simulink model "FMS"  (R2018b)
settings: configuration reference "fms_config" (kept outside this file)
values from neighbouring files (symbols this model uses):
  FMS_EXPORT = Simulink.Parameter(FMS_EXPORT_VALUE)    [fms_model_init.m]
  FMS_PARAM = Simulink.Parameter(FMS_PARAM_VALUE)    [fms_model_init.m]
undefined symbols (not defined in the file or in its folder): actuator_cmd, cmd_mask, ControlMode, ctrl_mode, DiscIntNeverNeededParam, FMS_Cmd, home, mode, PilotMode, r_cmd, reset, state, status, timestamp, u_cmd, VehicleState, VehicleStatus, wp_consume, wp_current
libraries: simulink x46, FMT_Model_Lib x35, hdlsllib x2
(part 2 of 3)

== system FMS/FMS Commander/Commander/Arm/Assist/Position/Velocity_Command/DeadZone ==
  u : Inport
  Dead Zone : DeadZone  LowerValue=-th  UpperValue=th  SaturateOnIntegerOverflow=on
  Gain : Gain  Gain=1/(1-th)
  y : Outport
  wires:
  Gain/1 -> y/1
  Dead Zone/1 -> Gain/1
  u/1 -> Dead Zone/1

== system FMS/FMS Commander/Commander/Arm/Assist/Stabilize/Heading Command/Controller ==
  motion_state : Inport
  In Bus Element : Inport  Port=2  PortName=FMS_In
  In Bus Element1 : Inport  Port=2  PortName=FMS_In
  Brake Control : Subsystem  TreatAsAtomicUnit=on
  Hold Control : Subsystem  TreatAsAtomicUnit=on
  Merge : Merge  Inputs=3
  Move Control : Subsystem  TreatAsAtomicUnit=on
  Switch Case : SwitchCase  CaseConditions={MotionState.Hold, MotionState.Brake, MotionState.Move}  ShowDefaultCase=off
  psi_rate_cmd_radPs : Outport
  wires:
  Move Control/1(psi_rate_cmd_radPs) -> Merge/3
  Hold Control/1(psi_rate_cmd_radPs) -> Merge/1
  In Bus Element/1 -> Hold Control/1(FMS_In)
  Switch Case/1 -> Hold Control/Action
  motion_state/1 -> Switch Case/1
  In Bus Element1/1 -> Move Control/1(FMS_In)
  Merge/1 -> psi_rate_cmd_radPs/1
  Switch Case/3 -> Move Control/Action
  Brake Control/1(psi_rate_cmd_radPs) -> Merge/2
  Switch Case/2 -> Brake Control/Action

== system FMS/FMS Commander/Commander/Arm/Assist/Stabilize/Heading Command/Detect Movement ==
  FMS_In : Inport
  Abs1 : Abs
  Abs2 : Abs
  Bus Selector1 : BusSelector  OutputSignals=Pilot_Cmd.stick_roll,Pilot_Cmd.stick_throttle
  Compare To Constant : simulink/Logic and Bit Operations/Compare To Constant  relop=>  const=0.1  OutDataTypeStr=boolean
  Compare To Constant1 : simulink/Logic and Bit Operations/Compare To Constant  relop=<=  const=0.15  OutDataTypeStr=boolean
  Logical Operator : Logic  Operator=OR  AllPortsSameDT=off  OutDataTypeStr=boolean
  Motion State : Stateflow chart  TreatAsAtomicUnit=on
  motion_state : Outport
  wires:
  FMS_In/1 -> Bus Selector1/1
  Compare To Constant/1 -> Logical Operator/1
  Abs1/1 -> Compare To Constant/1
  Motion State/1(state) -> motion_state/1  "pos_ms"
  Bus Selector1/1 -> Abs1/1  "<stick_roll>"
  Bus Selector1/2 -> Abs2/1  "<stick_throttle>"
  Abs2/1 -> Compare To Constant1/1
  Compare To Constant1/1 -> Logical Operator/2
  Logical Operator/1 -> Motion State/1(motion_req)

== system FMS/FMS Commander/Commander/Arm/Assist/Stabilize/Reset/DeadZone ==
  u : Inport
  Dead Zone : DeadZone  LowerValue=-th  UpperValue=th  SaturateOnIntegerOverflow=on
  Gain : Gain  Gain=1/(1-th)
  y : Outport
  wires:
  Gain/1 -> y/1
  Dead Zone/1 -> Gain/1
  u/1 -> Dead Zone/1

== system FMS/FMS Commander/Commander/Arm/Assist/Stabilize/Reset/DeadZone1 ==
  u : Inport
  Dead Zone : DeadZone  LowerValue=-th  UpperValue=th  SaturateOnIntegerOverflow=on
  Gain : Gain  Gain=1/(1-th)
  y : Outport
  wires:
  u/1 -> Dead Zone/1
  Dead Zone/1 -> Gain/1
  Gain/1 -> y/1

== system FMS/FMS Commander/Commander/Arm/Auto/Mission/Mission_SubSystem/Velocity Commander ==
  p1 : Inport
  p2 : Inport  Port=2
  p3 : Inport  Port=3
  L1 : Inport  Port=4
  In Bus Element : Inport  Port=5  PortName=FMS_In  Element=INS_Out.vn
  In Bus Element1 : Inport  Port=5  PortName=FMS_In  Element=INS_Out.ve
  AccToRate : Gain  Gain=FMS_PARAM.AY_P
  L1 Reference WP : Subsystem
  Lateral Acceleration : Subsystem
  Mux1 : Mux  Inputs=2
  r_cmd : Outport
  wires:
  p3/1 -> Lateral Acceleration/3(p3), L1 Reference WP/3(P3)
  In Bus Element1/1 -> Mux1/2
  Mux1/1 -> Lateral Acceleration/1(Vg)
  p2/1 -> L1 Reference WP/2(P2)
  Lateral Acceleration/1(l1_a_cmd) -> AccToRate/1
  In Bus Element/1 -> Mux1/1
  L1 Reference WP/1(L1_WP) -> Lateral Acceleration/2(L1_WP)  "L1_WP"
  p1/1 -> L1 Reference WP/1(P1)
  L1/1 -> L1 Reference WP/4(L1), Lateral Acceleration/4(L1)
  AccToRate/1 -> r_cmd/1

== system FMS/FMS Commander/Commander/Arm/Auto/Mission/Mission_SubSystem/Way Points ==
  note: P1: path start point
      | P2: path end point
      | P3: vehicle point
  FMS_In : Inport
  Bus Selector : BusSelector  OutputSignals=INS_Out.x_R,INS_Out.y_R
  Bus Selector1 : BusSelector  OutputSignals=Cmd_In.sp_waypoint
  Bus Selector2 : BusSelector  OutputSignals=Cmd_In.cur_waypoint
  Mux : Mux  Inputs=2
  Reshape : Reshape  OutputDimensionality=Customize  OutputDimensions=[2,1]
  Reshape1 : Reshape  OutputDimensionality=Customize  OutputDimensions=[2,1]
  Reshape2 : Reshape  OutputDimensionality=Customize  OutputDimensions=[2,1]
  Selector : Selector  InputPortWidth=3  IndexOptions=Index vector (dialog)  Indices=[1 2]  OutputSizes=1
  Selector1 : Selector  InputPortWidth=3  IndexOptions=Index vector (dialog)  Indices=[1 2]  OutputSizes=1
  p1 : Outport
  p2 : Outport  Port=2
  p3 : Outport  Port=3
  wires:
  Reshape2/1 -> p3/1
  Reshape1/1 -> p1/1
  Reshape/1 -> p2/1
  Bus Selector/2 -> Mux/2  "<y_R>"
  Bus Selector/1 -> Mux/1  "<x_R>"
  FMS_In/1 -> Bus Selector2/1, Bus Selector1/1, Bus Selector/1
  Bus Selector1/1 -> Selector/1  "<sp_waypoint>"
  Selector/1 -> Reshape/1
  Bus Selector2/1 -> Selector1/1  "<cur_waypoint>"
  Mux/1 -> Reshape2/1
  Selector1/1 -> Reshape1/1

== system FMS/FMS Commander/Commander/Arm/Auto/Offboard/Velocity Rotation Command/Heading_Control ==
  FMS_In : Inport
  Bus Selector1 : BusSelector  OutputSignals=Auto_Cmd.psi_cmd
  Bus Selector2 : BusSelector  OutputSignals=INS_Out.psi
  Gain2 : Gain  Gain=FMS_PARAM.YAW_P  OutDataTypeStr=single
  Sum : Sum  Inputs=-+|
  psi_err_saturation : Subsystem
  heading_r_cmd : Outport
  wires:
  Sum/1 -> psi_err_saturation/1(psi_err_in)  "psi_error_rad"
  psi_err_saturation/1(psi_err_rad) -> Gain2/1
  Gain2/1 -> heading_r_cmd/1
  FMS_In/1 -> Bus Selector1/1, Bus Selector2/1
  Bus Selector2/1 -> Sum/1  "<psi>"
  Bus Selector1/1 -> Sum/2  "<psi_cmd>"

== system FMS/FMS Commander/Commander/Arm/Auto/Offboard/Velocity Rotation Command/Position Data ==
  FMS_In : Inport
  Bus Selector : BusSelector  OutputSignals=INS_Out.x_R,INS_Out.y_R
  Mux : Mux  Inputs=2
  Position Command : Subsystem
  Reshape : Reshape  OutputDimensionality=Customize  OutputDimensions=[2,1]
  Reshape1 : Reshape  OutputDimensionality=Customize  OutputDimensions=[2,1]
  pos_R : Outport
  pos_cmd : Outport  Port=2
  wires:
  Reshape1/1 -> pos_R/1
  Reshape/1 -> pos_cmd/1
  Bus Selector/2 -> Mux/2  "<y_R>"
  Bus Selector/1 -> Mux/1  "<x_R>"
  FMS_In/1 -> Position Command/1(FMS_In), Bus Selector/1
  Position Command/1(pos_O_cmd) -> Reshape/1
  Mux/1 -> Reshape1/1

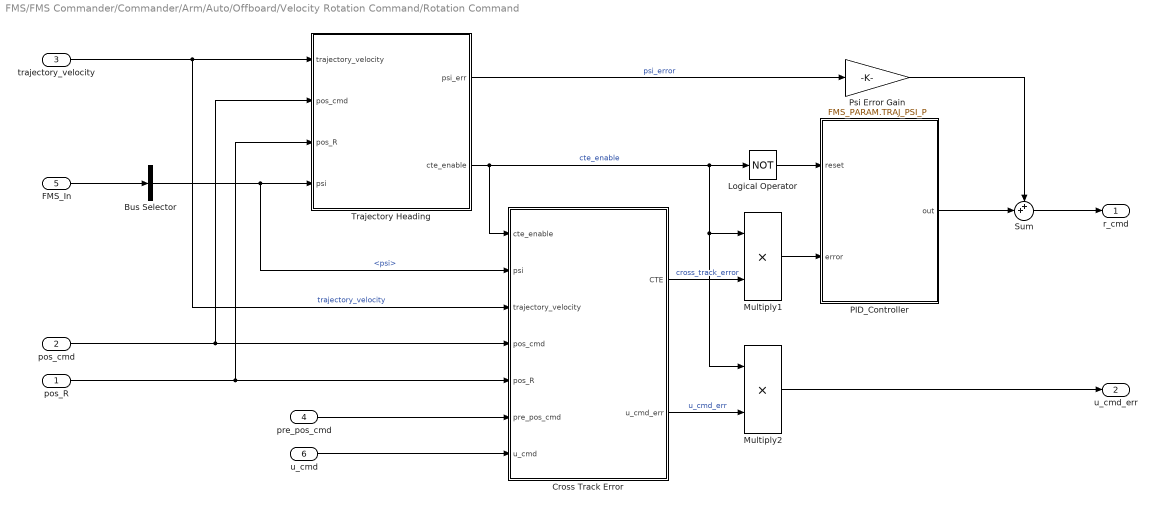
== system FMS/FMS Commander/Commander/Arm/Auto/Offboard/Velocity Rotation Command/Rotation Command ==
  pos_R : Inport
  pos_cmd : Inport  Port=2
  trajectory_velocity : Inport  Port=3
  pre_pos_cmd : Inport  Port=4
  FMS_In : Inport  Port=5
  u_cmd : Inport  Port=6
  Bus Selector : BusSelector  OutputSignals=INS_Out.psi
  Cross Track Error : Subsystem
  Logical Operator : Logic  Operator=NOT  AllPortsSameDT=off  OutDataTypeStr=boolean
  Multiply1 : Product
  Multiply2 : Product
  PID_Controller : Subsystem
  Psi Error Gain : Gain  Gain=FMS_PARAM.TRAJ_PSI_P  OutDataTypeStr=Inherit: Same as input
  Sum : Sum  Inputs=++|
  Trajectory Heading : Subsystem
  r_cmd : Outport
  u_cmd_err : Outport  Port=2
  wires:
  pos_cmd/1 -> Trajectory Heading/2(pos_cmd), Cross Track Error/4(pos_cmd)
  trajectory_velocity/1 -> Cross Track Error/3(trajectory_velocity), Trajectory Heading/1(trajectory_velocity)  "trajectory_velocity"
  pos_R/1 -> Trajectory Heading/3(pos_R), Cross Track Error/5(pos_R)
  Bus Selector/1 -> Trajectory Heading/4(psi), Cross Track Error/2(psi)  "<psi>"
  Cross Track Error/1(CTE) -> Multiply1/2  "cross_track_error"
  Psi Error Gain/1 -> Sum/1
  u_cmd/1 -> Cross Track Error/7(u_cmd)
  FMS_In/1 -> Bus Selector/1
  pre_pos_cmd/1 -> Cross Track Error/6(pre_pos_cmd)
  Cross Track Error/2(u_cmd_err) -> Multiply2/2  "u_cmd_err"
  Multiply2/1 -> u_cmd_err/1
  PID_Controller/1(out) -> Sum/2
  Sum/1 -> r_cmd/1
  Trajectory Heading/1(psi_err) -> Psi Error Gain/1  "psi_error"
  Trajectory Heading/2(cte_enable) -> Cross Track Error/1(cte_enable), Logical Operator/1, Multiply2/1, Multiply1/1  "cte_enable"
  Multiply1/1 -> PID_Controller/2(error)
  Logical Operator/1 -> PID_Controller/1(reset)

== system FMS/FMS Commander/Commander/Arm/Auto/Offboard/Velocity Rotation Command/Signal_Route ==
  FMS_In : Inport
  heading_r_cmd : Inport  Port=2
  pos_r_cmd : Inport  Port=3
  Bus Selector : BusSelector  OutputSignals=Auto_Cmd.cmd_mask
  Bus Selector1 : BusSelector  OutputSignals=Auto_Cmd.r_cmd
  Switch : Switch  Criteria=u2 > Threshold
  Switch1 : Switch  Criteria=u2 > Threshold
  psi_cmd_valid : simulink/Logic and Bit Operations/Bitwise Operator  logicop=AND  UseBitMask=on  BitMask=bin2dec('100000')  BitMaskRealWorld=Stored Integer
  r_cmd_valid : simulink/Logic and Bit Operations/Bitwise Operator  logicop=AND  UseBitMask=on  BitMask=bin2dec('100')  BitMaskRealWorld=Stored Integer
  r_cmd : Outport
  wires:
  FMS_In/1 -> Bus Selector1/1, Bus Selector/1
  pos_r_cmd/1 -> Switch1/3
  r_cmd_valid/1 -> Switch/2
  Bus Selector1/1 -> Switch/1  "<r_cmd>"
  Switch/1 -> r_cmd/1
  Bus Selector/1 -> psi_cmd_valid/1, r_cmd_valid/1  "<cmd_mask>"
  psi_cmd_valid/1 -> Switch1/2
  heading_r_cmd/1 -> Switch1/1
  Switch1/1 -> Switch/3

== system FMS/FMS Commander/Commander/Arm/Auto/Offboard/Velocity Rotation Command/Trajectory Velocity ==
  pos_cmd : Inport  OutDataTypeStr=single  PortDimensions=[2 1]
  pos_R : Inport  Port=2
  FMS_In : Inport  Port=3
  Bus Selector : BusSelector  OutputSignals=Auto_Cmd.timestamp
  Divide : Product  Inputs=*/
  Low Pass Filter : Subsystem
  Previous Pos Cmd : Subsystem
  Sum : Sum  Inputs=+-|
  dT Estimator : Subsystem
  trajectory_velocity : Outport  OutDataTypeStr=single  PortDimensions=[2 1]  VectorParamsAs1DForOutWhenUnconnected=on
  pre_pos_cmd : Outport  Port=2  OutDataTypeStr=single  PortDimensions=[2 1]  VectorParamsAs1DForOutWhenUnconnected=on
  wires:
  Low Pass Filter/1(y) -> trajectory_velocity/1
  Divide/1 -> Low Pass Filter/1(u)
  Sum/1 -> Divide/1
  pos_cmd/1 -> Sum/1, Previous Pos Cmd/1(pos_cmd)  "pos_cmd"
  pos_R/1 -> Previous Pos Cmd/2(pos_R)
  Previous Pos Cmd/1(prev_pos_cmd) -> pre_pos_cmd/1, Sum/2  "pre_pos_cmd"
  FMS_In/1 -> Bus Selector/1
  Bus Selector/1 -> dT Estimator/1(timestamp)  "<timestamp>"
  dT Estimator/1(dT) -> Divide/2  "dT"

== system FMS/FMS Commander/Commander/Arm/Auto/Offboard/Velocity Rotation Command/Velocity Command ==
  note: u command is always in body frame for car
  trajectory_velocity : Inport
  FMS_In : Inport  Port=2
  Bus Selector1 : BusSelector  OutputSignals=Auto_Cmd.cmd_mask
  Bus Selector2 : BusSelector  OutputSignals=Auto_Cmd.u_cmd
  Compare To Zero2 : simulink/Logic and Bit Operations/Compare To Zero  relop=>  OutDataTypeStr=boolean
  Saturation1 : Saturate  UpperLimit=FMS_PARAM.MAX_VEL  LowerLimit=0
  Switch : Switch  Criteria=u2 > Threshold
  Vector Modulus : FMT_Model_Lib/Math/Vector Modulus
      settings: SourceProductName=FMT Toolbox
  u_cmd valid : simulink/Logic and Bit Operations/Bitwise Operator  logicop=AND  UseBitMask=on  BitMask=bin2dec('10000000000000')  BitMaskRealWorld=Stored Integer
  u_cmd_C : Outport
  wires:
  Compare To Zero2/1 -> Switch/2
  Bus Selector2/1 -> Switch/1  "<u_cmd>"
  Saturation1/1 -> Switch/3
  Switch/1 -> u_cmd_C/1
  Bus Selector1/1 -> u_cmd valid/1  "<cmd_mask>"
  u_cmd valid/1 -> Compare To Zero2/1
  FMS_In/1 -> Bus Selector1/1, Bus Selector2/1
  trajectory_velocity/1 -> Vector Modulus/1
  Vector Modulus/1 -> Saturation1/1  "trajectory_speed"

== system FMS/FMS Commander/Commander/Arm/SubMode/Return/Velocity Commander/L1 Reference WP ==
  P1 : Inport
  P2 : Inport  Port=2
  P3 : Inport  Port=3
  L1 : Inport  Port=4
  Compare To Constant : simulink/Logic and Bit Operations/Compare To Constant  relop=>=  const=0  OutDataTypeStr=boolean
  Compare To Constant1 : simulink/Logic and Bit Operations/Compare To Constant  relop=>  const=0  OutDataTypeStr=boolean
  NearbyRefWP : MATLAB Function  TreatAsAtomicUnit=on
  OutRegionRegWP : MATLAB Function  TreatAsAtomicUnit=on
  Reshape : Reshape  OutputDimensionality=Customize  OutputDimensions=[2,1]
  SearchL1RefWP : MATLAB Function  TreatAsAtomicUnit=on
  Switch : Switch  Criteria=u2 > Threshold
  Switch1 : Switch  Criteria=u2 > Threshold
  L1_WP : Outport
  wires:
  Reshape/1 -> L1_WP/1
  Compare To Constant/1 -> Switch/2
  NearbyRefWP/2(d) -> Compare To Constant1/1  "distance"
  SearchL1RefWP/2(u) -> Compare To Constant/1  "l1_u"
  Compare To Constant1/1 -> Switch1/2
  P1/1 -> SearchL1RefWP/1(P1), OutRegionRegWP/1(P1)
  P2/1 -> SearchL1RefWP/2(P2), NearbyRefWP/1(P2), OutRegionRegWP/2(P2)
  P3/1 -> NearbyRefWP/2(P3), SearchL1RefWP/3(P3), OutRegionRegWP/3(P3)
  Switch/1 -> Switch1/3
  L1/1 -> SearchL1RefWP/4(L1), NearbyRefWP/3(L1)
  OutRegionRegWP/1(P) -> Switch/3  "out_WP"
  Switch1/1 -> Reshape/1
  SearchL1RefWP/1(P) -> Switch/1  "L1_Ref_P"
  NearbyRefWP/1(P) -> Switch1/1  "NearbyWP"

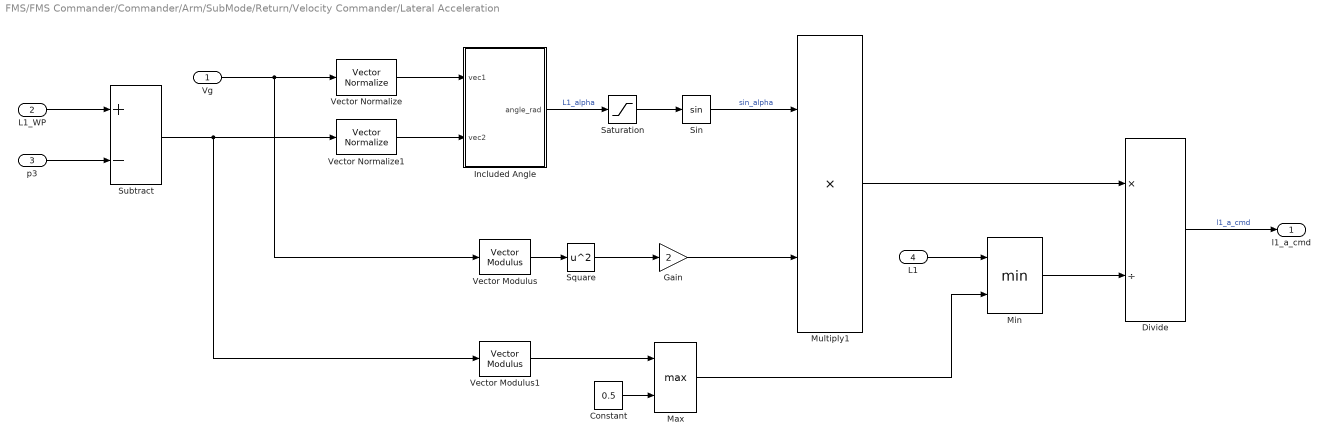
== system FMS/FMS Commander/Commander/Arm/SubMode/Return/Velocity Commander/Lateral Acceleration ==
  Vg : Inport
  L1_WP : Inport  Port=2
  p3 : Inport  Port=3
  L1 : Inport  Port=4
  Constant : Constant  Value=0.5  OutDataTypeStr=Inherit: Inherit via back propagation
  Divide : Product  Inputs=*/
  Gain : Gain  Gain=2
  Included Angle : Subsystem
  Max : MinMax  Function=max  Inputs=2
  Min : MinMax  Inputs=2
  Multiply1 : Product
  Saturation : Saturate  UpperLimit=pi/2  LowerLimit=-pi/2
  Sin : Trigonometry
  Square : Math  Operator=square  SaturateOnIntegerOverflow=on
  Subtract : Sum  Inputs=+-
  Vector Modulus : FMT_Model_Lib/Math/Vector Modulus
      settings: SourceProductName=FMT Toolbox
  Vector Modulus1 : FMT_Model_Lib/Math/Vector Modulus
      settings: SourceProductName=FMT Toolbox
  Vector Normalize : FMT_Model_Lib/Math/Vector Normalize
      settings: SourceProductName=FMT Toolbox
  Vector Normalize1 : FMT_Model_Lib/Math/Vector Normalize
      settings: SourceProductName=FMT Toolbox
  l1_a_cmd : Outport
  wires:
  Saturation/1 -> Sin/1
  Included Angle/1(angle_rad) -> Saturation/1  "L1_alpha"
  Vector Modulus/1 -> Square/1
  Subtract/1 -> Vector Modulus1/1, Vector Normalize1/1
  Gain/1 -> Multiply1/2
  L1_WP/1 -> Subtract/1
  Vector Normalize/1 -> Included Angle/1(vec1)
  Multiply1/1 -> Divide/1
  Divide/1 -> l1_a_cmd/1  "l1_a_cmd"
  Vector Normalize1/1 -> Included Angle/2(vec2)
  Square/1 -> Gain/1
  L1/1 -> Min/1
  Vg/1 -> Vector Normalize/1, Vector Modulus/1
  Sin/1 -> Multiply1/1  "sin_alpha"
  p3/1 -> Subtract/2
  Vector Modulus1/1 -> Max/1
  Constant/1 -> Max/2
  Max/1 -> Min/2
  Min/1 -> Divide/2

== system FMS/FMS Commander/Commander/Arm/Assist/Position/Position Command/Controller/Brake Control ==
  Action Port : ActionPort  InitializeStates=reset  ActionType=case
  Constant : Constant  Value=0  OutDataTypeStr=single
  r_cmd_radPs : Outport
  wires:
  Constant/1 -> r_cmd_radPs/1

== system FMS/FMS Commander/Commander/Arm/Assist/Position/Position Command/Controller/Hold Control ==
  FMS_In : Inport
  u_cmd : Inport  Port=2
  Action Port : ActionPort  InitializeStates=reset  ActionType=case
  AccToRate : Gain  Gain=FMS_PARAM.AY_P
  Bus Selector1 : BusSelector  OutputSignals=INS_Out.vn,INS_Out.ve
  FMS_In1 : InportShadow
  L1 : Constant  Value=FMS_PARAM.L1  OutDataTypeStr=single
  L1_Reference_WP : Subsystem
  Lateral_Acceleration : Subsystem
  Mux : Mux  Inputs=2
  Path_Ray : Subsystem
  r_cmd_radPs : Outport
  wires:
  FMS_In/1 -> Path_Ray/1(FMS_In)
  Path_Ray/1(p_vehicle) -> Lateral_Acceleration/1(p_vehicle), L1_Reference_WP/1(c)
  Path_Ray/2(p_0) -> L1_Reference_WP/2(p_0)
  Path_Ray/3(n) -> L1_Reference_WP/3(n)
  L1/1 -> L1_Reference_WP/4(L1), Lateral_Acceleration/3(L1)
  FMS_In1/1 -> Bus Selector1/1
  Bus Selector1/1 -> Mux/1  "<vn>"
  Bus Selector1/2 -> Mux/2  "<ve>"
  L1_Reference_WP/1(L1_WP) -> Lateral_Acceleration/2(L1_WP)
  Mux/1 -> Lateral_Acceleration/4(Vg)
  Lateral_Acceleration/1(ay_cmd_mPs2) -> AccToRate/1
  AccToRate/1 -> r_cmd_radPs/1
  u_cmd/1 -> Path_Ray/2(u_cmd)

== system FMS/FMS Commander/Commander/Arm/Assist/Position/Position Command/Controller/Move Control ==
  FMS_In : Inport
  Action Port : ActionPort  InitializeStates=reset  ActionType=case
  Bus Selector : BusSelector  OutputSignals=Pilot_Cmd.stick_roll
  DeadZone : Subsystem  mask{th=0.1}
      mask prompts: th "Threshold"
      mask Display: disp('Dead Zone')
  Gain6 : Gain  Gain=FMS_PARAM.MAX_R  OutDataTypeStr=single
  r_cmd_radPs : Outport
  wires:
  Bus Selector/1 -> DeadZone/1(u)  "<stick_roll>"
  Gain6/1 -> r_cmd_radPs/1
  FMS_In/1 -> Bus Selector/1
  DeadZone/1(y) -> Gain6/1

== system FMS/FMS Commander/Commander/Arm/Assist/Stabilize/Heading Command/Controller/Brake Control ==
  Action Port : ActionPort  InitializeStates=reset  ActionType=case
  Constant : Constant  Value=0  OutDataTypeStr=single
  psi_rate_cmd_radPs : Outport
  wires:
  Constant/1 -> psi_rate_cmd_radPs/1

== system FMS/FMS Commander/Commander/Arm/Assist/Stabilize/Heading Command/Controller/Hold Control ==
  FMS_In : Inport
  Action Port : ActionPort  InitializeStates=reset  ActionType=case
  Bus_Selection : Subsystem
  Delay : Delay  DelayLength=1  InitialConditionSource=Input port
      settings: InputPortMap=u0,p4
  Gain2 : Gain  Gain=FMS_PARAM.YAW_P  OutDataTypeStr=single
  Sum : Sum  Inputs=-+|
  psi_err_saturation : Subsystem
  psi_rate_cmd_radPs : Outport
  wires:
  FMS_In/1 -> Bus_Selection/1(FMS_In)
  Gain2/1 -> psi_rate_cmd_radPs/1
  psi_err_saturation/1(psi_err_rad) -> Gain2/1
  Sum/1 -> psi_err_saturation/1(psi_err_in)  "psi_error_rad"
  Delay/1 -> Sum/2, Delay/1  "psi_cmd_rad"
  Bus_Selection/1(psi_rad) -> Delay/2, Sum/1  "psi_est_rad"

== system FMS/FMS Commander/Commander/Arm/Assist/Stabilize/Heading Command/Controller/Move Control ==
  FMS_In : Inport
  Action Port : ActionPort  InitializeStates=reset  ActionType=case
  Bus Selector : BusSelector  OutputSignals=Pilot_Cmd.stick_roll
  DeadZone : Subsystem  mask{th=0.1}
      mask prompts: th "Threshold"
      mask Display: disp('Dead Zone')
  Gain : Gain  Gain=FMS_PARAM.MAX_R
  psi_rate_cmd_radPs : Outport
  wires:
  Bus Selector/1 -> DeadZone/1(u)  "<stick_roll>"
  FMS_In/1 -> Bus Selector/1
  DeadZone/1(y) -> Gain/1
  Gain/1 -> psi_rate_cmd_radPs/1

== system FMS/FMS Commander/Commander/Arm/Auto/Mission/Mission_SubSystem/Velocity Commander/L1 Reference WP ==
  P1 : Inport
  P2 : Inport  Port=2
  P3 : Inport  Port=3
  L1 : Inport  Port=4
  Compare To Constant : simulink/Logic and Bit Operations/Compare To Constant  relop=>=  const=0  OutDataTypeStr=boolean
  Compare To Constant1 : simulink/Logic and Bit Operations/Compare To Constant  relop=>  const=0  OutDataTypeStr=boolean
  NearbyRefWP : MATLAB Function  TreatAsAtomicUnit=on
  OutRegionRegWP : MATLAB Function  TreatAsAtomicUnit=on
  Reshape : Reshape  OutputDimensionality=Customize  OutputDimensions=[2,1]
  SearchL1RefWP : MATLAB Function  TreatAsAtomicUnit=on
  Switch : Switch  Criteria=u2 > Threshold
  Switch1 : Switch  Criteria=u2 > Threshold
  L1_WP : Outport
  wires:
  Reshape/1 -> L1_WP/1
  Compare To Constant/1 -> Switch/2
  NearbyRefWP/2(d) -> Compare To Constant1/1  "distance"
  SearchL1RefWP/2(u) -> Compare To Constant/1  "l1_u"
  Compare To Constant1/1 -> Switch1/2
  P1/1 -> SearchL1RefWP/1(P1), OutRegionRegWP/1(P1)
  P2/1 -> SearchL1RefWP/2(P2), NearbyRefWP/1(P2), OutRegionRegWP/2(P2)
  P3/1 -> NearbyRefWP/2(P3), SearchL1RefWP/3(P3), OutRegionRegWP/3(P3)
  Switch/1 -> Switch1/3
  L1/1 -> SearchL1RefWP/4(L1), NearbyRefWP/3(L1)
  OutRegionRegWP/1(P) -> Switch/3  "out_WP"
  Switch1/1 -> Reshape/1
  SearchL1RefWP/1(P) -> Switch/1  "L1_Ref_P"
  NearbyRefWP/1(P) -> Switch1/1  "NearbyWP"

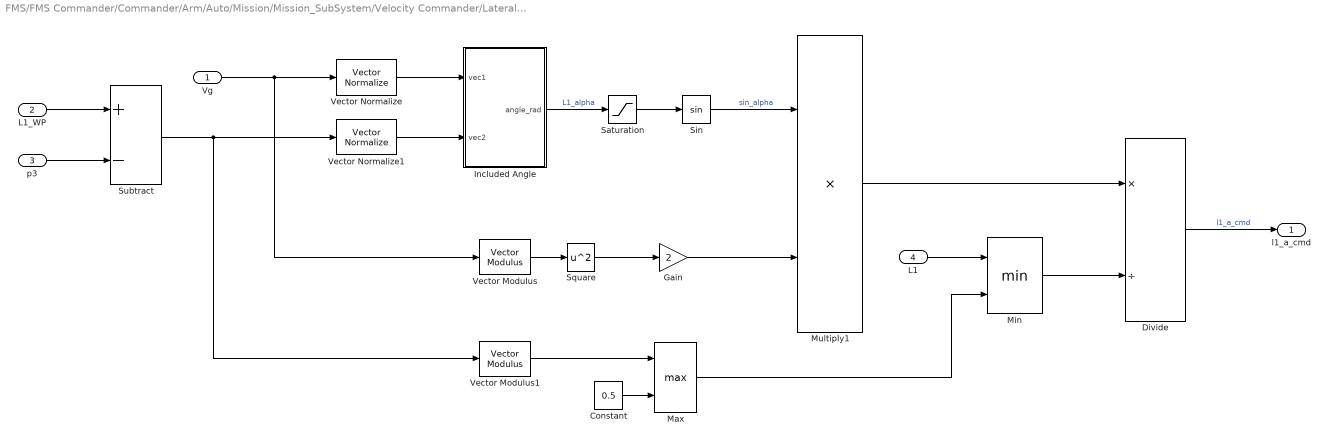
== system FMS/FMS Commander/Commander/Arm/Auto/Mission/Mission_SubSystem/Velocity Commander/Lateral Acceleration ==
  Vg : Inport
  L1_WP : Inport  Port=2
  p3 : Inport  Port=3
  L1 : Inport  Port=4
  Constant : Constant  Value=0.5  OutDataTypeStr=Inherit: Inherit via back propagation
  Divide : Product  Inputs=*/
  Gain : Gain  Gain=2
  Included Angle : Subsystem
  Max : MinMax  Function=max  Inputs=2
  Min : MinMax  Inputs=2
  Multiply1 : Product
  Saturation : Saturate  UpperLimit=pi/2  LowerLimit=-pi/2
  Sin : Trigonometry
  Square : Math  Operator=square  SaturateOnIntegerOverflow=on
  Subtract : Sum  Inputs=+-
  Vector Modulus : FMT_Model_Lib/Math/Vector Modulus
      settings: SourceProductName=FMT Toolbox
  Vector Modulus1 : FMT_Model_Lib/Math/Vector Modulus
      settings: SourceProductName=FMT Toolbox
  Vector Normalize : FMT_Model_Lib/Math/Vector Normalize
      settings: SourceProductName=FMT Toolbox
  Vector Normalize1 : FMT_Model_Lib/Math/Vector Normalize
      settings: SourceProductName=FMT Toolbox
  l1_a_cmd : Outport
  wires:
  Saturation/1 -> Sin/1
  Included Angle/1(angle_rad) -> Saturation/1  "L1_alpha"
  Vector Modulus/1 -> Square/1
  Subtract/1 -> Vector Modulus1/1, Vector Normalize1/1
  Gain/1 -> Multiply1/2
  L1_WP/1 -> Subtract/1
  Vector Normalize/1 -> Included Angle/1(vec1)
  Multiply1/1 -> Divide/1
  Divide/1 -> l1_a_cmd/1  "l1_a_cmd"
  Vector Normalize1/1 -> Included Angle/2(vec2)
  Square/1 -> Gain/1
  L1/1 -> Min/1
  Vg/1 -> Vector Normalize/1, Vector Modulus/1
  Sin/1 -> Multiply1/1  "sin_alpha"
  p3/1 -> Subtract/2
  Vector Modulus1/1 -> Max/1
  Constant/1 -> Max/2
  Max/1 -> Min/2
  Min/1 -> Divide/2

== system FMS/FMS Commander/Commander/Arm/Auto/Offboard/Velocity Rotation Command/Heading_Control/psi_err_saturation ==
  psi_err_in : Inport
  Abs : Abs
  Compare To Constant : simulink/Logic and Bit Operations/Compare To Constant  relop=>  const=pi  OutDataTypeStr=boolean
  Constant : Constant  Value=2*pi  OutDataTypeStr=single
  Multiply : Product
  Sign : Signum
  Subtract : Sum  Inputs=-+
  Switch : Switch  Criteria=u2 > Threshold
  psi_err_rad : Outport
  wires:
  Multiply/1 -> Switch/1
  Sign/1 -> Multiply/2
  Subtract/1 -> Multiply/1
  Constant/1 -> Subtract/1
  Switch/1 -> psi_err_rad/1
  Compare To Constant/1 -> Switch/2
  Abs/1 -> Compare To Constant/1, Subtract/2
  psi_err_in/1 -> Abs/1, Switch/3, Sign/1

== system FMS/FMS Commander/Commander/Arm/Auto/Offboard/Velocity Rotation Command/Position Data/Position Command ==
  FMS_In : Inport
  Body_FRD : Subsystem
  Bus Selector : BusSelector  OutputSignals=INS_Out
  Bus Selector2 : BusSelector  OutputSignals=Auto_Cmd.frame
  Command_Mask : Subsystem
  Global_NED : Subsystem
  Index Vector : MultiPortSwitch  DataPortOrder=Zero-based contiguous  Inputs=4  zeroidx=on
  Local_FRD : Subsystem
  Local_NED : Subsystem
  Position_Command : Subsystem
  Selector : Selector  InputPortWidth=3  IndexOptions=Index vector (dialog)  Indices=[1 2]  OutputSizes=1
  pos_O_cmd : Outport
  wires:
  Position_Command/1(pos_cmd_R) -> Local_FRD/1(pos_R_cmd), Body_FRD/2(pos_B_cmd), Local_NED/1(pos_R_cmd), Global_NED/1(pos_O_cmd)
  Bus Selector/1 -> Body_FRD/1(INS_Out)  "<INS_Out>"
  Bus Selector2/1 -> Index Vector/1  "<frame>"
  FMS_In/1 -> Position_Command/1(FMS_In), Bus Selector2/1, Bus Selector/1, Command_Mask/1(FMS_In)
  Command_Mask/1(pos_mask) -> Body_FRD/3(pos_mask), Local_FRD/2(pos_mask), Local_NED/2(pos_mask), Global_NED/2(pos_mask)
  Global_NED/1(pos_cmd) -> Index Vector/2
  Index Vector/1 -> Selector/1
  Body_FRD/1(pos_O_cmd) -> Index Vector/5
  Local_FRD/1(pos_O_cmd) -> Index Vector/4
  Local_NED/1(pos_O_cmd) -> Index Vector/3
  Selector/1 -> pos_O_cmd/1

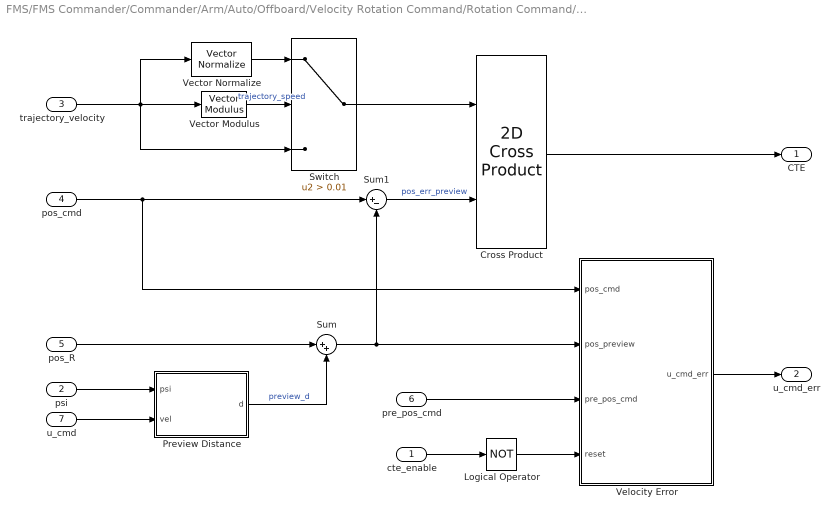
== system FMS/FMS Commander/Commander/Arm/Auto/Offboard/Velocity Rotation Command/Rotation Command/Cross Track Error ==
  cte_enable : Inport
  psi : Inport  Port=2
  trajectory_velocity : Inport  Port=3  OutDataTypeStr=single
  pos_cmd : Inport  Port=4  OutDataTypeStr=single  PortDimensions=[2 1]
  pos_R : Inport  Port=5  OutDataTypeStr=single  PortDimensions=[2 1]
  pre_pos_cmd : Inport  Port=6
  u_cmd : Inport  Port=7
  Cross Product : FMT_Model_Lib/Math/2D Cross Product
      settings: SourceProductName=FMT Toolbox
  Logical Operator : Logic  Operator=NOT  AllPortsSameDT=off  OutDataTypeStr=boolean
  Preview Distance : Subsystem
  Sum : Sum  Inputs=|++
  Sum1 : Sum  Inputs=|+-
  Switch : Switch  Criteria=u2 > Threshold  Threshold=0.01
  Vector Modulus : FMT_Model_Lib/Math/Vector Modulus
      settings: SourceProductName=FMT Toolbox
  Vector Normalize : FMT_Model_Lib/Math/Vector Normalize
      settings: SourceProductName=FMT Toolbox
  Velocity Error : Subsystem
  CTE : Outport  OutDataTypeStr=single  PortDimensions=1  VectorParamsAs1DForOutWhenUnconnected=on
  u_cmd_err : Outport  Port=2  OutDataTypeStr=single  PortDimensions=1  VectorParamsAs1DForOutWhenUnconnected=on
  wires:
  Cross Product/1 -> CTE/1
  pos_R/1 -> Sum/1
  psi/1 -> Preview Distance/1(psi)
  u_cmd/1 -> Preview Distance/2(vel)
  Preview Distance/1(d) -> Sum/2  "preview_d"
  Sum/1 -> Velocity Error/2(pos_preview), Sum1/2
  Sum1/1 -> Cross Product/2  "pos_err_preview"
  pre_pos_cmd/1 -> Velocity Error/3(pre_pos_cmd)
  Velocity Error/1(u_cmd_err) -> u_cmd_err/1
  pos_cmd/1 -> Sum1/1, Velocity Error/1(pos_cmd)
  Vector Modulus/1 -> Switch/2  "trajectory_speed"
  Switch/1 -> Cross Product/1
  trajectory_velocity/1 -> Vector Normalize/1, Switch/3, Vector Modulus/1
  Vector Normalize/1 -> Switch/1
  Logical Operator/1 -> Velocity Error/4(reset)
  cte_enable/1 -> Logical Operator/1

== system FMS/FMS Commander/Commander/Arm/Auto/Offboard/Velocity Rotation Command/Rotation Command/PID_Controller ==
  reset : Inport
  error : Inport  Port=2
  Add : Sum  Inputs=+++
  D_Control : Subsystem  mask{kd=FMS_PARAM.TRAJ_CTE_D, max_d=pi/10, min_d=-pi/10}
  I_Control : Subsystem  mask{ki=FMS_PARAM.TRAJ_CTE_I, max_i=pi/5, min_i=-pi/5}
  P_Control : Subsystem  mask{kp=FMS_PARAM.TRAJ_CTE_P}
  out : Outport
  wires:
  Add/1 -> out/1
  reset/1 -> D_Control/2(reset), I_Control/2(reset)
  D_Control/1(d_out) -> Add/3  "cte_d_out"
  I_Control/1(i_out) -> Add/2  "cte_i_out"
  P_Control/1(p_out) -> Add/1  "cte_p_out"
  error/1 -> D_Control/1(err), I_Control/1(err), P_Control/1(err)

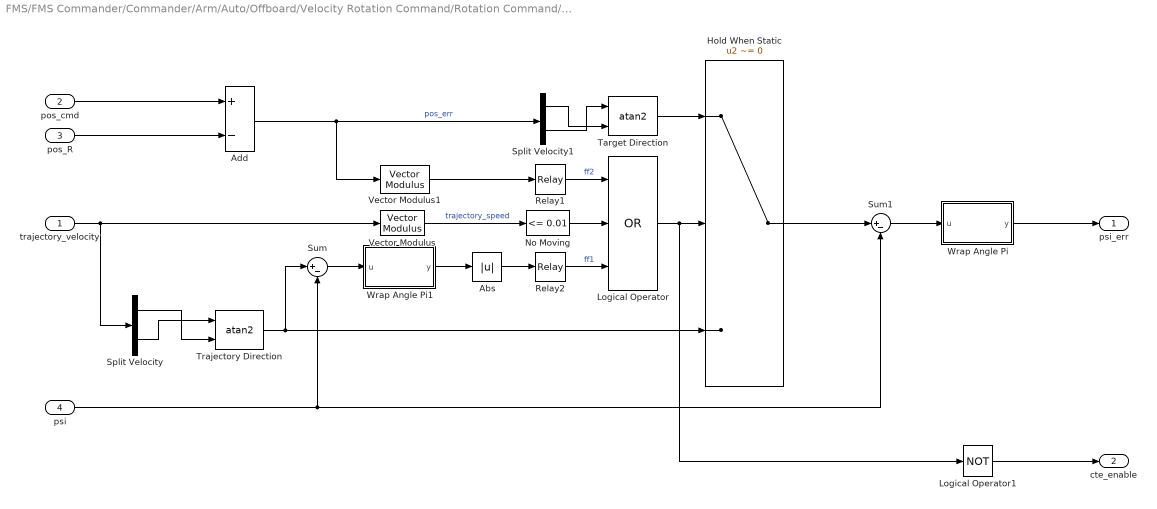
== system FMS/FMS Commander/Commander/Arm/Auto/Offboard/Velocity Rotation Command/Rotation Command/Trajectory Heading ==
  trajectory_velocity : Inport  OutDataTypeStr=single  PortDimensions=[2 1]
  pos_cmd : Inport  Port=2
  pos_R : Inport  Port=3
  psi : Inport  Port=4
  Abs : Abs
  Add : Sum  Inputs=+-
  Hold When Static : Switch  Criteria=u2 ~= 0
  Logical Operator : Logic  Operator=OR  Inputs=3  AllPortsSameDT=off  OutDataTypeStr=boolean
  Logical Operator1 : Logic  Operator=NOT  AllPortsSameDT=off  OutDataTypeStr=boolean
  No Moving : simulink/Logic and Bit Operations/Compare To Constant  relop=<=  const=0.01  OutDataTypeStr=boolean
  Relay1 : Relay  OnSwitchValue=2  OffSwitchValue=1
  Relay2 : Relay  OnSwitchValue=pi/2  OffSwitchValue=pi/4
  Split Velocity : Demux  Outputs=2
  Split Velocity1 : Demux  Outputs=2
  Sum : Sum  Inputs=|+-
  Sum1 : Sum  Inputs=|+-
  Target Direction : Trigonometry  Operator=atan2
  Trajectory Direction : Trigonometry  Operator=atan2
  Vector Modulus : FMT_Model_Lib/Math/Vector Modulus
      settings: SourceProductName=FMT Toolbox
  Vector Modulus1 : FMT_Model_Lib/Math/Vector Modulus
      settings: SourceProductName=FMT Toolbox
  Wrap Angle Pi : Subsystem
  Wrap Angle Pi1 : Subsystem
  psi_err : Outport
  cte_enable : Outport  Port=2
  wires:
  Trajectory Direction/1 -> Sum/1, Hold When Static/3
  No Moving/1 -> Logical Operator/2
  Split Velocity/2 -> Trajectory Direction/1
  Split Velocity/1 -> Trajectory Direction/2
  Vector Modulus/1 -> No Moving/1  "trajectory_speed"
  trajectory_velocity/1 -> Split Velocity/1, Vector Modulus/1
  Split Velocity1/1 -> Target Direction/2
  Split Velocity1/2 -> Target Direction/1
  Add/1 -> Vector Modulus1/1, Split Velocity1/1  "pos_err"
  pos_cmd/1 -> Add/1
  pos_R/1 -> Add/2
  Target Direction/1 -> Hold When Static/1
  psi/1 -> Sum1/2, Sum/2
  Sum1/1 -> Wrap Angle Pi/1(u)
  Hold When Static/1 -> Sum1/1
  Wrap Angle Pi1/1(y) -> Abs/1
  Abs/1 -> Relay2/1
  Sum/1 -> Wrap Angle Pi1/1(u)
  Relay2/1 -> Logical Operator/3  "ff1"
  Vector Modulus1/1 -> Relay1/1
  Relay1/1 -> Logical Operator/1  "ff2"
  Logical Operator/1 -> Logical Operator1/1, Hold When Static/2
  Wrap Angle Pi/1(y) -> psi_err/1
  Logical Operator1/1 -> cte_enable/1

== system FMS/FMS Commander/Commander/Arm/Auto/Offboard/Velocity Rotation Command/Trajectory Velocity/Low Pass Filter ==
  u : Inport  OutDataTypeStr=single
  Blend : Sum
  Filter Coefficient : Gain  Gain=0.0769230769230769  OutDataTypeStr=Inherit: Same as input
  One Minus Filter Coefficient : Gain  Gain=0.923076923076923  OutDataTypeStr=Inherit: Same as input
  Previous Output : UnitDelay  SampleTime=-1
  y : Outport  OutDataTypeStr=single  VectorParamsAs1DForOutWhenUnconnected=on
  wires:
  Blend/1 -> y/1, Previous Output/1
  Filter Coefficient/1 -> Blend/1
  Previous Output/1 -> One Minus Filter Coefficient/1
  One Minus Filter Coefficient/1 -> Blend/2
  u/1 -> Filter Coefficient/1

== system FMS/FMS Commander/Commander/Arm/Auto/Offboard/Velocity Rotation Command/Trajectory Velocity/Previous Pos Cmd ==
  pos_cmd : Inport
  pos_R : Inport  Port=2
  Delay : Delay  DelayLength=1  InitialConditionSource=Input port
      settings: InputPortMap=u0,p4
  Detect Change : simulink/Logic and Bit Operations/Detect Change  vinit=0  OutDataTypeStr=boolean
  Logical Operator : Logic  Operator=OR  Inputs=1  AllPortsSameDT=off  OutDataTypeStr=boolean
  Previous Position Command : Delay  DelayLength=1
  Switch : Switch  Criteria=u2 > Threshold
  prev_pos_cmd : Outport
  wires:
  Detect Change/1 -> Logical Operator/1
  pos_R/1 -> Delay/2
  Previous Position Command/1 -> Switch/3
  pos_cmd/1 -> Detect Change/1, Delay/1
  Delay/1 -> Switch/1
  Logical Operator/1 -> Switch/2
  Switch/1 -> Previous Position Command/1, prev_pos_cmd/1

== system FMS/FMS Commander/Commander/Arm/Auto/Offboard/Velocity Rotation Command/Trajectory Velocity/dT Estimator ==
  timestamp : Inport
  Add : Sum  Inputs=-+
  Delay1 : Delay  DelayLength=1
  Delta Time : Delay  DelayLength=1
  Detect Change1 : simulink/Logic and Bit Operations/Detect Change  vinit=0  OutDataTypeStr=boolean
  Saturation : Saturate  UpperLimit=10000  LowerLimit=FMS_EXPORT.period
  Switch3 : Switch  Criteria=u2 > Threshold
  ms_to_second : Gain  Gain=0.001  OutDataTypeStr=single
  dT : Outport
  wires:
  Detect Change1/1 -> Switch3/2
  Add/1 -> Switch3/1
  Saturation/1 -> Delta Time/1, ms_to_second/1
  Delta Time/1 -> Switch3/3
  timestamp/1 -> Delay1/1, Add/2, Detect Change1/1
  Switch3/1 -> Saturation/1
  ms_to_second/1 -> dT/1
  Delay1/1 -> Add/1

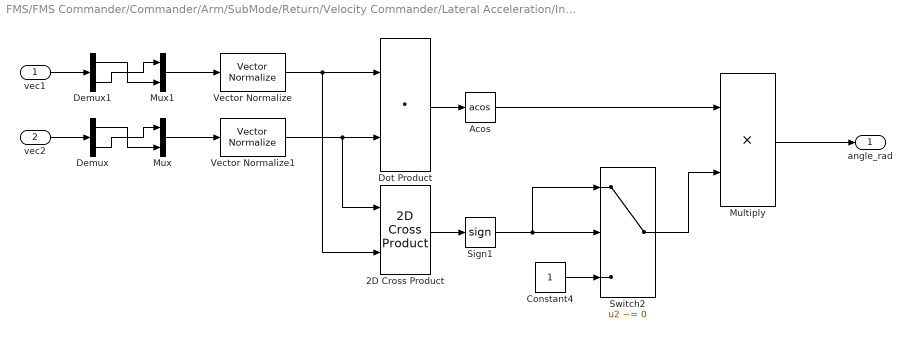
== system FMS/FMS Commander/Commander/Arm/SubMode/Return/Velocity Commander/Lateral Acceleration/Included Angle ==
  vec1 : Inport
  vec2 : Inport  Port=2
  2D Cross Product : FMT_Model_Lib/Math/2D Cross Product
      settings: SourceProductName=FMT Toolbox
  Acos : Trigonometry  Operator=acos
  Constant4 : Constant  OutDataTypeStr=single
  Demux : Demux  Outputs=2
  Demux1 : Demux  Outputs=2
  Dot Product : DotProduct  InputSameDT=on  OutDataTypeStr=Inherit: Inherit via internal rule
  Multiply : Product
  Mux : Mux  Inputs=2
  Mux1 : Mux  Inputs=2
  Sign1 : Signum
  Switch2 : Switch  Criteria=u2 ~= 0
  Vector Normalize : FMT_Model_Lib/Math/Vector Normalize
      settings: SourceProductName=FMT Toolbox
  Vector Normalize1 : FMT_Model_Lib/Math/Vector Normalize
      settings: SourceProductName=FMT Toolbox
  angle_rad : Outport
  wires:
  Switch2/1 -> Multiply/2
  Acos/1 -> Multiply/1
  Mux/1 -> Vector Normalize1/1
  vec2/1 -> Demux/1
  Constant4/1 -> Switch2/3
  Demux/1 -> Mux/2
  vec1/1 -> Demux1/1
  Multiply/1 -> angle_rad/1
  2D Cross Product/1 -> Sign1/1
  Vector Normalize/1 -> 2D Cross Product/2, Dot Product/1
  Demux/2 -> Mux/1
  Vector Normalize1/1 -> 2D Cross Product/1, Dot Product/2
  Sign1/1 -> Switch2/2, Switch2/1
  Demux1/2 -> Mux1/1
  Mux1/1 -> Vector Normalize/1
  Demux1/1 -> Mux1/2
  Dot Product/1 -> Acos/1

== system FMS/FMS Commander/Commander/Arm/Assist/Position/Position Command/Controller/Hold Control/L1_Reference_WP ==
  c : Inport
  p_0 : Inport  Port=2
  n : Inport  Port=3
  L1 : Inport  Port=4
  Compare To Zero : simulink/Logic and Bit Operations/Compare To Zero  relop=>  OutDataTypeStr=boolean
  OutRegionRefWP : MATLAB Function  TreatAsAtomicUnit=on
  SearchL1RefWP : MATLAB Function  TreatAsAtomicUnit=on
  Switch : Switch  Criteria=u2 > Threshold
  L1_WP : Outport
  wires:
  c/1 -> OutRegionRefWP/1(c), SearchL1RefWP/1(c)
  p_0/1 -> OutRegionRefWP/2(p0), SearchL1RefWP/2(p0)
  n/1 -> OutRegionRefWP/3(n), SearchL1RefWP/3(n)  "L1_n"
  L1/1 -> SearchL1RefWP/4(L1)
  SearchL1RefWP/1(P) -> Switch/1
  SearchL1RefWP/2(t) -> Compare To Zero/1  "L1_t"
  Compare To Zero/1 -> Switch/2
  OutRegionRefWP/1(P) -> Switch/3
  Switch/1 -> L1_WP/1  "L1_WP"

== system FMS/FMS Commander/Commander/Arm/Assist/Position/Position Command/Controller/Hold Control/Lateral_Acceleration ==
  p_vehicle : Inport
  L1_WP : Inport  Port=2
  L1 : Inport  Port=3
  Vg : Inport  Port=4
  L1_Lateral_Acceleration : Subsystem
  Subtract : Sum  Inputs=+-
  ay_cmd_mPs2 : Outport
  wires:
  L1_WP/1 -> Subtract/1  "l1_wp2"
  p_vehicle/1 -> Subtract/2
  L1/1 -> L1_Lateral_Acceleration/1(L1)
  Vg/1 -> L1_Lateral_Acceleration/2(Vg)
  Subtract/1 -> L1_Lateral_Acceleration/3(l1_path)  "l1_path"
  L1_Lateral_Acceleration/1(l1_a_cmd) -> ay_cmd_mPs2/1  "gg1"

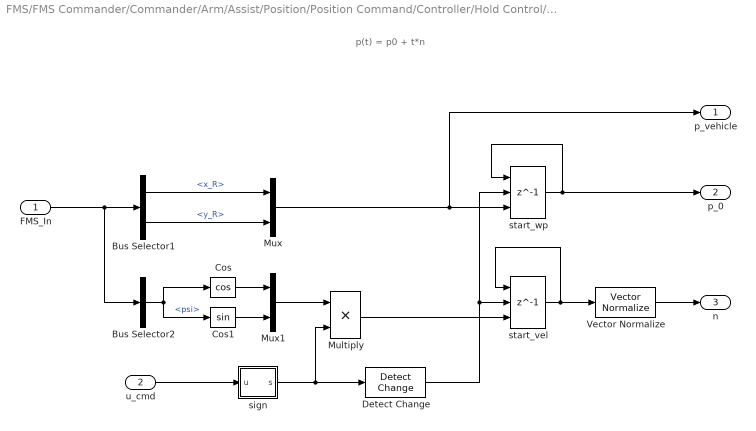
== system FMS/FMS Commander/Commander/Arm/Assist/Position/Position Command/Controller/Hold Control/Path_Ray ==
  note: p(t) = p0 + t*n
  FMS_In : Inport
  u_cmd : Inport  Port=2
  Bus Selector1 : BusSelector  OutputSignals=INS_Out.x_R,INS_Out.y_R
  Bus Selector2 : BusSelector  OutputSignals=INS_Out.psi
  Cos : Trigonometry  Operator=cos
  Cos1 : Trigonometry
  Detect Change : simulink/Logic and Bit Operations/Detect Change  vinit=0  OutDataTypeStr=boolean
  Multiply : Product
  Mux : Mux  Inputs=2
  Mux1 : Mux  Inputs=2
  Vector Normalize : FMT_Model_Lib/Math/Vector Normalize
      settings: SourceProductName=FMT Toolbox
  sign : Subsystem
  start_vel : Delay  DelayLength=1  InitialConditionSource=Input port  ExternalReset=Rising
      settings: InputPortMap=u0,r5,p4
  start_wp : Delay  DelayLength=1  InitialConditionSource=Input port  ExternalReset=Rising
      settings: InputPortMap=u0,r5,p4
  p_vehicle : Outport
  p_0 : Outport  Port=2
  n : Outport  Port=3
  wires:
  Bus Selector1/2 -> Mux/2  "<y_R>"
  Mux/1 -> p_vehicle/1, start_wp/3
  start_wp/1 -> start_wp/1, p_0/1
  Bus Selector1/1 -> Mux/1  "<x_R>"
  start_vel/1 -> start_vel/1, Vector Normalize/1
  Vector Normalize/1 -> n/1
  FMS_In/1 -> Bus Selector2/1, Bus Selector1/1
  Detect Change/1 -> start_wp/2, start_vel/2
  Cos/1 -> Mux1/1
  Bus Selector2/1 -> Cos1/1, Cos/1  "<psi>"
  Cos1/1 -> Mux1/2
  u_cmd/1 -> sign/1(u)
  sign/1(s) -> Multiply/2, Detect Change/1
  Mux1/1 -> Multiply/1
  Multiply/1 -> start_vel/3

== system FMS/FMS Commander/Commander/Arm/Assist/Position/Position Command/Controller/Move Control/DeadZone ==
  u : Inport
  Dead Zone : DeadZone  LowerValue=-th  UpperValue=th  SaturateOnIntegerOverflow=on
  Gain : Gain  Gain=1/(1-th)
  y : Outport
  wires:
  Gain/1 -> y/1
  Dead Zone/1 -> Gain/1
  u/1 -> Dead Zone/1

== system FMS/FMS Commander/Commander/Arm/Assist/Stabilize/Heading Command/Controller/Hold Control/Bus_Selection ==
  FMS_In : Inport
  Bus Selector2 : BusSelector  OutputSignals=INS_Out.psi
  psi_rad : Outport
  wires:
  Bus Selector2/1 -> psi_rad/1  "<psi>"
  FMS_In/1 -> Bus Selector2/1

== system FMS/FMS Commander/Commander/Arm/Assist/Stabilize/Heading Command/Controller/Hold Control/psi_err_saturation ==
  psi_err_in : Inport
  Abs : Abs
  Compare To Constant : simulink/Logic and Bit Operations/Compare To Constant  relop=>  const=pi  OutDataTypeStr=boolean
  Constant : Constant  Value=2*pi  OutDataTypeStr=single
  Multiply : Product
  Sign : Signum
  Subtract : Sum  Inputs=-+
  Switch : Switch  Criteria=u2 > Threshold
  psi_err_rad : Outport
  wires:
  Multiply/1 -> Switch/1
  Sign/1 -> Multiply/2
  Subtract/1 -> Multiply/1
  Constant/1 -> Subtract/1
  Switch/1 -> psi_err_rad/1
  Compare To Constant/1 -> Switch/2
  Abs/1 -> Compare To Constant/1, Subtract/2
  psi_err_in/1 -> Abs/1, Switch/3, Sign/1

== system FMS/FMS Commander/Commander/Arm/Assist/Stabilize/Heading Command/Controller/Move Control/DeadZone ==
  u : Inport
  Dead Zone : DeadZone  LowerValue=-th  UpperValue=th  SaturateOnIntegerOverflow=on
  Gain : Gain  Gain=1/(1-th)
  y : Outport
  wires:
  Gain/1 -> y/1
  Dead Zone/1 -> Gain/1
  u/1 -> Dead Zone/1

== system FMS/FMS Commander/Commander/Arm/Auto/Mission/Mission_SubSystem/Velocity Commander/Lateral Acceleration/Included Angle ==
  vec1 : Inport
  vec2 : Inport  Port=2
  2D Cross Product : FMT_Model_Lib/Math/2D Cross Product
      settings: SourceProductName=FMT Toolbox
  Acos : Trigonometry  Operator=acos
  Constant4 : Constant  OutDataTypeStr=single
  Demux : Demux  Outputs=2
  Demux1 : Demux  Outputs=2
  Dot Product : DotProduct  InputSameDT=on  OutDataTypeStr=Inherit: Inherit via internal rule
  Multiply : Product
  Mux : Mux  Inputs=2
  Mux1 : Mux  Inputs=2
  Sign1 : Signum
  Switch2 : Switch  Criteria=u2 ~= 0
  Vector Normalize : FMT_Model_Lib/Math/Vector Normalize
      settings: SourceProductName=FMT Toolbox
  Vector Normalize1 : FMT_Model_Lib/Math/Vector Normalize
      settings: SourceProductName=FMT Toolbox
  angle_rad : Outport
  wires:
  Switch2/1 -> Multiply/2
  Acos/1 -> Multiply/1
  Mux/1 -> Vector Normalize1/1
  vec2/1 -> Demux/1
  Constant4/1 -> Switch2/3
  Demux/1 -> Mux/2
  vec1/1 -> Demux1/1
  Multiply/1 -> angle_rad/1
  2D Cross Product/1 -> Sign1/1
  Vector Normalize/1 -> 2D Cross Product/2, Dot Product/1
  Demux/2 -> Mux/1
  Vector Normalize1/1 -> 2D Cross Product/1, Dot Product/2
  Sign1/1 -> Switch2/2, Switch2/1
  Demux1/2 -> Mux1/1
  Mux1/1 -> Vector Normalize/1
  Demux1/1 -> Mux1/2
  Dot Product/1 -> Acos/1

== system FMS/FMS Commander/Commander/Arm/Auto/Offboard/Velocity Rotation Command/Position Data/Position Command/Body_FRD ==
  INS_Out : Inport
  pos_B_cmd : Inport  Port=2
  pos_mask : Inport  Port=3
  Bus Selector : BusSelector  OutputSignals=psi
  Bus Selector1 : BusSelector  OutputSignals=x_R,y_R,h_R
  Gain : Gain  Gain=-1
  Multiply : Product
  Multiply1 : Product  Multiplication=Matrix(*)
  Mux : Mux  Inputs=3
  Psi To DCM : FMT_Model_Lib/Transformation/Psi To DCM
      settings: SourceProductName=FMT Toolbox
  Sum : Sum  Inputs=++|
  Transpose : Math  Operator=transpose  SaturateOnIntegerOverflow=on
  pos_O_cmd : Outport
  wires:
  Psi To DCM/1 -> Transpose/1
  INS_Out/1 -> Bus Selector/1, Bus Selector1/1
  Multiply/1 -> Multiply1/2
  pos_mask/1 -> Multiply/2
  Transpose/1 -> Multiply1/1  "M_OC"
  pos_B_cmd/1 -> Multiply/1
  Multiply1/1 -> Sum/2
  Sum/1 -> pos_O_cmd/1
  Mux/1 -> Sum/1
  Bus Selector/1 -> Psi To DCM/1  "<psi>"
  Bus Selector1/1 -> Mux/1  "<x_R>"
  Bus Selector1/2 -> Mux/2  "<y_R>"
  Bus Selector1/3 -> Gain/1  "<h_R>"
  Gain/1 -> Mux/3

== system FMS/FMS Commander/Commander/Arm/Auto/Offboard/Velocity Rotation Command/Position Data/Position Command/Command_Mask ==
  FMS_In : Inport
  Bus Selector3 : BusSelector  OutputSignals=Auto_Cmd.cmd_mask
  Compare To Zero : simulink/Logic and Bit Operations/Compare To Zero  relop=>  OutDataTypeStr=boolean
  Compare To Zero1 : simulink/Logic and Bit Operations/Compare To Zero  relop=>  OutDataTypeStr=boolean
  Logical Operator : Logic  Operator=OR  AllPortsSameDT=off  OutDataTypeStr=boolean
  Mux : Mux  Inputs=3
  Mux3 : Mux  Inputs=3
  alt_cmd valid : simulink/Logic and Bit Operations/Bitwise Operator  logicop=AND  UseBitMask=on  BitMask=bin2dec('1000000000000')  BitMaskRealWorld=Stored Integer
  lat_cmd valid : simulink/Logic and Bit Operations/Bitwise Operator  logicop=AND  UseBitMask=on  BitMask=bin2dec('10000000000')  BitMaskRealWorld=Stored Integer
  lon_cmd valid : simulink/Logic and Bit Operations/Bitwise Operator  logicop=AND  UseBitMask=on  BitMask=bin2dec('100000000000')  BitMaskRealWorld=Stored Integer
  x_cmd valid : simulink/Logic and Bit Operations/Bitwise Operator  logicop=AND  UseBitMask=on  BitMask=bin2dec('10000000')  BitMaskRealWorld=Stored Integer
  y_cmd valid : simulink/Logic and Bit Operations/Bitwise Operator  logicop=AND  UseBitMask=on  BitMask=bin2dec('100000000')  BitMaskRealWorld=Stored Integer
  z_cmd valid : simulink/Logic and Bit Operations/Bitwise Operator  logicop=AND  UseBitMask=on  BitMask=bin2dec('1000000000')  BitMaskRealWorld=Stored Integer
  pos_mask : Outport
  wires:
  FMS_In/1 -> Bus Selector3/1
  x_cmd valid/1 -> Mux/1
  z_cmd valid/1 -> Mux/3
  y_cmd valid/1 -> Mux/2
  Mux/1 -> Compare To Zero/1
  lon_cmd valid/1 -> Mux3/2
  alt_cmd valid/1 -> Mux3/3
  Mux3/1 -> Compare To Zero1/1
  lat_cmd valid/1 -> Mux3/1
  Bus Selector3/1 -> y_cmd valid/1, x_cmd valid/1, z_cmd valid/1, lat_cmd valid/1, lon_cmd valid/1, alt_cmd valid/1  "<cmd_mask>"
  Compare To Zero1/1 -> Logical Operator/2
  Compare To Zero/1 -> Logical Operator/1
  Logical Operator/1 -> pos_mask/1

== system FMS/FMS Commander/Commander/Arm/Auto/Offboard/Velocity Rotation Command/Position Data/Position Command/Global_NED ==
  pos_O_cmd : Inport
  pos_mask : Inport  Port=2
  Multiply : Product
  pos_cmd : Outport
  wires:
  pos_O_cmd/1 -> Multiply/1
  Multiply/1 -> pos_cmd/1
  pos_mask/1 -> Multiply/2

== system FMS/FMS Commander/Commander/Arm/Auto/Offboard/Velocity Rotation Command/Position Data/Position Command/Local_FRD ==
  pos_R_cmd : Inport
  pos_mask : Inport  Port=2
  Data Store Read : DataStoreRead  DataStoreName=home
  Home Position : Subsystem
  Multiply : Product
  Multiply3 : Product  Multiplication=Matrix(*)
  Psi To DCM2 : FMT_Model_Lib/Transformation/Psi To DCM
      settings: SourceProductName=FMT Toolbox
  Selector : Selector  InputPortWidth=4  IndexOptions=Index vector (dialog)  Indices=4  OutputSizes=1
  Sum : Sum  Inputs=++|
  Transpose : Math  Operator=transpose  SaturateOnIntegerOverflow=on
  pos_O_cmd : Outport
  wires:
  Multiply/1 -> Multiply3/2
  pos_mask/1 -> Multiply/2
  Psi To DCM2/1 -> Transpose/1
  Transpose/1 -> Multiply3/1  "M_OC"
  Selector/1 -> Psi To DCM2/1
  Data Store Read/1 -> Home Position/1(home), Selector/1
  pos_R_cmd/1 -> Multiply/1
  Multiply3/1 -> Sum/2
  Sum/1 -> pos_O_cmd/1
  Home Position/1(home_pos) -> Sum/1

== system FMS/FMS Commander/Commander/Arm/Auto/Offboard/Velocity Rotation Command/Position Data/Position Command/Local_NED ==
  pos_R_cmd : Inport
  pos_mask : Inport  Port=2
  Data Store Read : DataStoreRead  DataStoreName=home
  Home Position : Subsystem
  Multiply : Product
  Sum : Sum  Inputs=++|
  pos_O_cmd : Outport
  wires:
  Sum/1 -> pos_O_cmd/1
  pos_R_cmd/1 -> Multiply/1
  pos_mask/1 -> Multiply/2
  Multiply/1 -> Sum/2
  Data Store Read/1 -> Home Position/1(home)
  Home Position/1(home_pos) -> Sum/1

== system FMS/FMS Commander/Commander/Arm/Auto/Offboard/Velocity Rotation Command/Position Data/Position Command/Position_Command ==
  FMS_In : Inport
  Command_Mask : Subsystem
  Global_Position_Command : Subsystem
  Local_Position_Command : Subsystem
  Switch : Switch  Criteria=u2 > Threshold
  pos_cmd_R : Outport
  wires:
  FMS_In/1 -> Local_Position_Command/1(FMS_In), Command_Mask/1(FMS_In), Global_Position_Command/1(FMS_In)
  Switch/1 -> pos_cmd_R/1
  Local_Position_Command/1(pos_cmd_R) -> Switch/3
  Global_Position_Command/1(pos_cmd_O) -> Switch/1
  Command_Mask/1(global_cmd_valid) -> Switch/2

== system FMS/FMS Commander/Commander/Arm/Auto/Offboard/Velocity Rotation Command/Rotation Command/Cross Track Error/Preview Distance ==
  psi : Inport
  vel : Inport  Port=2
  Cos1 : Trigonometry  Operator=cos
  Multiply : Product
  Sin1 : Trigonometry
  T : Gain  Gain=FMS_PARAM.TRAJ_PREVIEW_T
  Tangent Vector1 : Mux  Inputs=2
  d : Outport
  wires:
  T/1 -> Multiply/2
  vel/1 -> T/1
  psi/1 -> Sin1/1, Cos1/1
  Tangent Vector1/1 -> Multiply/1  "forward direction"
  Cos1/1 -> Tangent Vector1/1
  Sin1/1 -> Tangent Vector1/2
  Multiply/1 -> d/1

== system FMS/FMS Commander/Commander/Arm/Auto/Offboard/Velocity Rotation Command/Rotation Command/Cross Track Error/Velocity Error ==
  pos_cmd : Inport
  pos_preview : Inport  Port=2
  pre_pos_cmd : Inport  Port=3
  reset : Inport  Port=4
  Add : Sum  Inputs=+-
  Add1 : Sum  Inputs=-+
  Add2 : Sum  Inputs=+-
  Dot Product : DotProduct  InputSameDT=on  OutDataTypeStr=Inherit: Inherit via internal rule
  Dot Product1 : DotProduct  InputSameDT=on  OutDataTypeStr=Inherit: Inherit via internal rule
  I_Control : Subsystem  mask{ki=FMS_PARAM.TRAJ_U_I, max_i=FMS_PARAM.TRAJ_U_I_MAX, min_i=FMS_PARAM.TRAJ_U_I_MIN}
  Multiply : Product
  Multiply1 : Product
  Sign : Signum
  Vector Modulus : FMT_Model_Lib/Math/Vector Modulus
      settings: SourceProductName=FMT Toolbox
  Vector Normalize : FMT_Model_Lib/Math/Vector Normalize
      settings: SourceProductName=FMT Toolbox
  u_cmd_err : Outport
  wires:
  pos_cmd/1 -> Add/1
  pre_pos_cmd/1 -> Add1/1, Add/2
  pos_preview/1 -> Add1/2
  Add/1 -> Dot Product1/1, Add2/1, Vector Normalize/1
  Add1/1 -> Dot Product/2
  Vector Normalize/1 -> Dot Product/1, Multiply/1
  Dot Product/1 -> Multiply/2
  Multiply/1 -> Add2/2
  Add2/1 -> Dot Product1/2, Vector Modulus/1
  Dot Product1/1 -> Sign/1
  Sign/1 -> Multiply1/1
  Vector Modulus/1 -> Multiply1/2
  reset/1 -> I_Control/2(reset)
  I_Control/1(i_out) -> u_cmd_err/1
  Multiply1/1 -> I_Control/1(err)

== system FMS/FMS Commander/Commander/Arm/Auto/Offboard/Velocity Rotation Command/Rotation Command/PID_Controller/D_Control ==
  err : Inport
  reset : Inport  Port=2
  DT Filter : FMT_Model_Lib/Filter/DT Filter  fc=20
      settings: SourceProductName=FMT Toolbox
  Multiply : Product  OutDataTypeStr=Inherit: Same as first input
  Saturation : Saturate  UpperLimit=max_d  LowerLimit=min_d
  gain1 : Constant  Value=kd  OutDataTypeStr=single
  d_out : Outport
  wires:
  DT Filter/1 -> Multiply/2
  gain1/1 -> Multiply/1
  reset/1 -> DT Filter/2
  Saturation/1 -> d_out/1
  Multiply/1 -> Saturation/1
  err/1 -> DT Filter/1

== system FMS/FMS Commander/Commander/Arm/Auto/Offboard/Velocity Rotation Command/Rotation Command/PID_Controller/I_Control ==
  err : Inport
  reset : Inport  Port=2
  Constant : Constant  Value=0  OutDataTypeStr=single
  Discrete-Time Integrator : DiscreteIntegrator  ExternalReset=level  InitialConditionSource=external  SampleTime=-1  LimitOutput=on  UpperSaturationLimit=max_i  LowerSaturationLimit=min_i  ICPrevOutput=DiscIntNeverNeededParam  ICPrevScaledInput=DiscIntNeverNeededParam
  Multiply : Product  OutDataTypeStr=Inherit: Same as first input
  gain1 : Constant  Value=ki  OutDataTypeStr=single
  i_out : Outport
  wires:
  Multiply/1 -> Discrete-Time Integrator/1
  gain1/1 -> Multiply/1
  Discrete-Time Integrator/1 -> i_out/1
  Constant/1 -> Discrete-Time Integrator/3
  reset/1 -> Discrete-Time Integrator/2
  err/1 -> Multiply/2

== system FMS/FMS Commander/Commander/Arm/Auto/Offboard/Velocity Rotation Command/Rotation Command/PID_Controller/P_Control ==
  err : Inport
  Multiply : Product  OutDataTypeStr=Inherit: Same as first input
  gain1 : Constant  Value=kp  OutDataTypeStr=single
  p_out : Outport
  wires:
  gain1/1 -> Multiply/1
  Multiply/1 -> p_out/1
  err/1 -> Multiply/2

== system FMS/FMS Commander/Commander/Arm/Auto/Offboard/Velocity Rotation Command/Rotation Command/Trajectory Heading/Wrap Angle Pi ==
  u : Inport  OutDataTypeStr=single  PortDimensions=1
  Direction : Signum
  Exceeds Pi : simulink/Logic and Bit Operations/Compare To Constant  relop=>  const=pi  OutDataTypeStr=boolean
  Magnitude : Abs
  Reduce By Two Pi : Sum  Inputs=+-
  Select Wrapped : Switch  Criteria=u2 ~= 0
  Signed Reduction : Product  Inputs=**
  Two Pi : Constant  Value=2*pi  OutDataTypeStr=single
  y : Outport  OutDataTypeStr=single  PortDimensions=1  VectorParamsAs1DForOutWhenUnconnected=on
  wires:
  Select Wrapped/1 -> y/1
  Exceeds Pi/1 -> Select Wrapped/2
  Two Pi/1 -> Reduce By Two Pi/2
  Reduce By Two Pi/1 -> Signed Reduction/2
  Direction/1 -> Signed Reduction/1
  Magnitude/1 -> Exceeds Pi/1, Reduce By Two Pi/1
  Signed Reduction/1 -> Select Wrapped/1
  u/1 -> Direction/1, Select Wrapped/3, Magnitude/1

== system FMS/FMS Commander/Commander/Arm/Auto/Offboard/Velocity Rotation Command/Rotation Command/Trajectory Heading/Wrap Angle Pi1 ==
  u : Inport  OutDataTypeStr=single  PortDimensions=1
  Direction : Signum
  Exceeds Pi : simulink/Logic and Bit Operations/Compare To Constant  relop=>  const=pi  OutDataTypeStr=boolean
  Magnitude : Abs
  Reduce By Two Pi : Sum  Inputs=+-
  Select Wrapped : Switch  Criteria=u2 ~= 0
  Signed Reduction : Product  Inputs=**
  Two Pi : Constant  Value=2*pi  OutDataTypeStr=single
  y : Outport  OutDataTypeStr=single  PortDimensions=1  VectorParamsAs1DForOutWhenUnconnected=on
  wires:
  Select Wrapped/1 -> y/1
  Exceeds Pi/1 -> Select Wrapped/2
  Two Pi/1 -> Reduce By Two Pi/2
  Reduce By Two Pi/1 -> Signed Reduction/2
  Direction/1 -> Signed Reduction/1
  Magnitude/1 -> Exceeds Pi/1, Reduce By Two Pi/1
  Signed Reduction/1 -> Select Wrapped/1
  u/1 -> Direction/1, Select Wrapped/3, Magnitude/1
